simulink model "second_order_discrete"  (R2025b)
settings: Solver=VariableStepAuto  StartTime=0.0  StopTime=5  FixedStep=0.001  RelTol=1e-3
InitFcn:
  | % % Tunable knob
  | % T_set = 200;
  | % s_CL = -6/T_set;
  | % % Kp = s_CL^2;
  | % % Kd = -2*s_CL;
  | %
  | % % Kp = 0.001064;
  | % % Kd = 0.063514;
  | %
  | % % Kp = 0.000537;
  | % % Kd = 0.038196;
  | %
  | % % Kp = 0.00045;
  | % % Kd = 0.040196;
  | %
  | %             Kp = 0.0003;
  | %             Kd = 0.09;
  | %
  | % Kob = 10;
  | %
  | % %             K = 164.458741/50*1;
  | % % tau1 = 160.525043;
  | % % tau2 = 835.747525;
  | % %             L_comp = 13.297226;
  | % %             L_sys  = 13.297226;
  | % K = 1.467057642011806*2;
  | % K0 = 1.467057642011806*2;
  | % tau1 = 5.108331033027039e+02;
  | % tau2 = 35.728915073943433;
  | % L_comp = 15.024369999999999;
  | % L_sys = 15.024369999999999;
  | % % K = 1.455368;
  | % % K0 = 1.455368;
  | % % tau1 = 18.226428;
  | % % tau2 = 538.493088;
  | % % L_comp = 33.344271;
  | % % L_sys = 33.344271;
  | % t1 = tau1*tau2;
  | % b0 = K0/t1;
  | %
  | % % Derived quantities
  | % s_ESO = Kob*s_CL;
  | % l1 = -3*s_ESO;
  | % l2 = 3*s_ESO^2;
  | % l3 = -s_ESO^3;
  | %
  | % A = [-l1  1  0;
  | %      -l2  0  1
  | %      -l3  0  0];
  | %
  | % B = [0   l1
  | %      b0  l2;
  | %      0   l3];
  | %
  | % % discrete equivalent
  | % Ts = 0.005;
  | % Ad = [1  Ts  Ts^2/2
  | %       0   1      Ts
  | %       0   0       1];
  | % Bd = [b0*Ts^2/2; b0*Ts; 0];
  | % z_ESO = exp(s_ESO*Ts);
  | % dl1 = 1-z_ESO^3;
  | % dl2 = 3/(2*Ts) * (1-z_ESO)^2*(1+z_ESO);
  | % dl3 = 1/Ts^2 * (1-z_ESO)^3;
  | % Cd = [1 0 0]; Ld = [dl1;dl2;dl3];
  | % Aeso = Ad - Ld*Cd*Ad;
  | % Beso = Bd - Ld*Cd*Bd;
  | % delay_comp = round(L_comp*200);
  | % delay_sys  = round(L_sys*200);
  | % K1 = Kp; K2 = Kd;
  | 
  | 
  | 
  | % Tunable knob
  | T_set = 200;
  | s_CL = -6/T_set;
  | % Kp = s_CL^2;
  | % Kd = -2*s_CL;
  | Kp = 0.00055;
  | Kd = 0.06;
  | 
  | Kob = 2;
  | 
  | K = 1.6937;
  | K0 = 1.6937 ;
  | tau1 = 792.76;
  | tau2 = 56.103;
  | L_comp = 29.97;
  | L_sys = 29.97;
  | t1 = tau1*tau2;
  | b0 = K0/t1;
  | 
  | % Derived quantities
  | s_ESO = Kob*s_CL;
  | l1 = -3*s_ESO;
  | l2 = 3*s_ESO^2;
  | l3 = -s_ESO^3;
  | 
  | A = [-l1  1  0;
  |      -l2  0  1
  |      -l3  0  0];
  | 
  | B = [0   l1
  |      b0  l2;
  |      0   l3];
  | 
  | % discrete equivalent
  | Ts = 0.005;
  | Ad = [1  Ts  Ts^2/2
  |       0   1      Ts
  |       0   0       1];
  | Bd = [b0*Ts^2/2; b0*Ts; 0];
  | z_ESO = exp(s_ESO*Ts);
  | dl1 = 1-z_ESO^3;
  | dl2 = 3/(2*Ts) * (1-z_ESO)^2*(1+z_ESO);
  | dl3 = 1/Ts^2 * (1-z_ESO)^3;
  | Cd = [1 0 0]; Ld = [dl1;dl2;dl3];
  | Aeso = Ad - Ld*Cd*Ad;
  | Beso = Bd - Ld*Cd*Bd;
  | delay_comp = round(L_comp*200);
  | delay_sys  = round(L_sys*200);
  | K1 = Kp; K2 = Kd;
libraries: simulink_extras x1
settings Model: Creator=SARIR  LastModifiedBy=MG8102
settings RTWCC: GPUComputeCapability=3.5

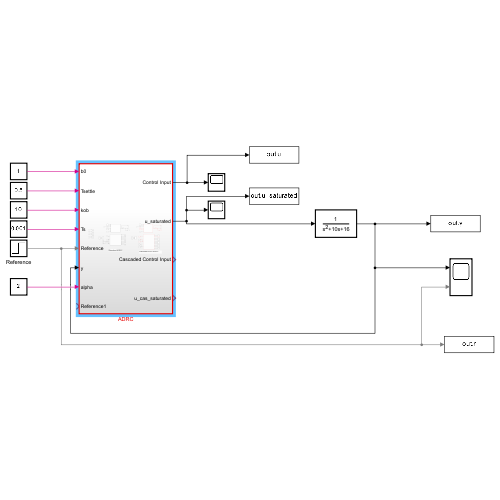
[thumbnail: Simulink's stored preview of the top-level diagram]
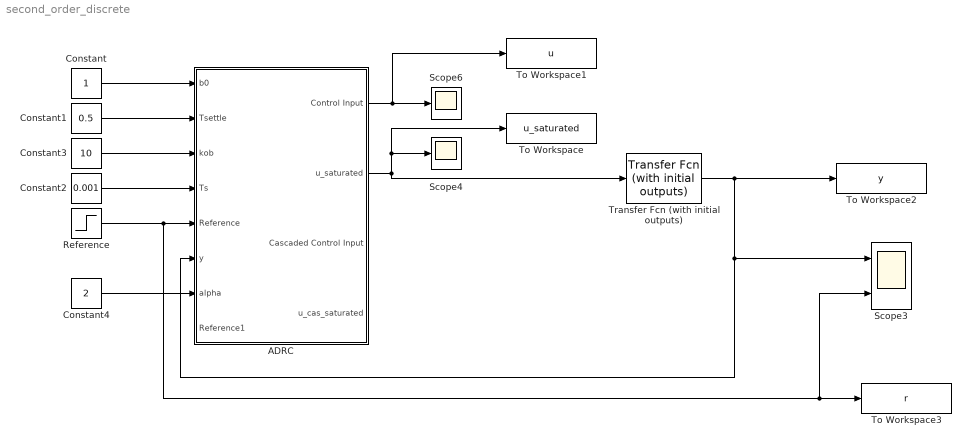
== system second_order_discrete ==
  ADRC : Subsystem
  Constant : Constant
  Constant1 : Constant  Value=0.5
  Constant2 : Constant  Value=0.001
  Constant3 : Constant  Value=10
  Constant4 : Constant  Value=2
  Reference : Step  Time=2  SampleTime=0
  Scope3 : Scope  NumInputPorts=2
      settings: ActiveDisplayYMinimum=-0.13260362865071351  ActiveDisplayYMaximum=1.1934326578564218
  Scope4 : Scope
      settings: ActiveDisplayYMinimum=-12.499999999999996  ActiveDisplayYMaximum=112.5  DataLoggingVariableName=ScopeData13
  Scope6 : Scope
      settings: ActiveDisplayYMinimum=-0.96663811924557952  ActiveDisplayYMaximum=8.8198546513386518  DataLoggingVariableName=ScopeData15
  To Workspace : ToWorkspace  VariableName=u_saturated  SaveFormat=Timeseries  SampleTime=-1
  To Workspace1 : ToWorkspace  VariableName=u  SaveFormat=Timeseries  SampleTime=-1
  To Workspace2 : ToWorkspace  VariableName=y  SaveFormat=Timeseries  SampleTime=-1
  To Workspace3 : ToWorkspace  VariableName=r  SaveFormat=Timeseries  SampleTime=-1
  Transfer Fcn (with initial outputs) : simulink_extras/Additional Linear/Transfer Fcn (with initial outputs)  N=[1]  D=[1 10 16]  Y0=0  U0=0
  wires:
  Reference/1 -> Scope3/2, To Workspace3/1, ADRC/5(Reference)
  Constant/1 -> ADRC/1(b0)
  Constant1/1 -> ADRC/2(Tsettle)
  Constant3/1 -> ADRC/3(kob)
  ADRC/1(Control Input) -> To Workspace1/1, Scope6/1
  ADRC/2(u_saturated) -> Scope4/1, To Workspace/1, Transfer Fcn (with initial outputs)/1
  Constant2/1 -> ADRC/4(Ts)
  Transfer Fcn (with initial outputs)/1 -> ADRC/6(y), Scope3/1, To Workspace2/1
  Constant4/1 -> ADRC/7(alpha)

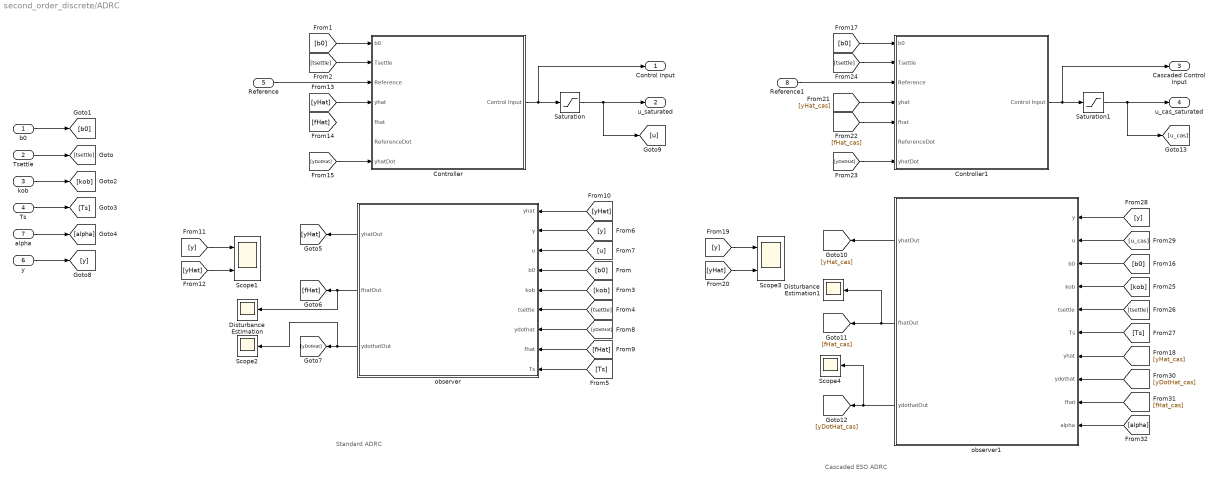
== system second_order_discrete/ADRC ==
  note: Standard ADRC
  note: Cascaded ESO ADRC
  b0 : Inport
  Tsettle : Inport  Port=2
  kob : Inport  Port=3
  Ts : Inport  Port=4
  Reference : Inport  Port=5
  y : Inport  Port=6
  alpha : Inport  Port=7
  Reference1 : Inport  Port=8
  Controller : Subsystem
  Controller1 : Subsystem
  Disturbance Estimation : Scope
      settings: ActiveDisplayYMinimum=-1  ActiveDisplayYMaximum=1  DataLoggingVariableName=ScopeData2
  Disturbance Estimation1 : Scope
      settings: ActiveDisplayYMinimum=-1  ActiveDisplayYMaximum=1  DataLoggingVariableName=ScopeData12
  Saturation : Saturate  UpperLimit=100  LowerLimit=0
  Saturation1 : Saturate  UpperLimit=100  LowerLimit=0
  Scope1 : Scope  NumInputPorts=2
      settings: ActiveDisplayYMinimum=-8.9116041220478586  ActiveDisplayYMaximum=80.204437098430745
  Scope2 : Scope
      settings: ActiveDisplayYMinimum=-1  ActiveDisplayYMaximum=1  DataLoggingVariableName=ScopeData2
  Scope3 : Scope  NumInputPorts=2
      settings: ActiveDisplayYMinimum=-8.9116041220478586  ActiveDisplayYMaximum=80.204437098430745  DataLoggingVariableName=ScopeData14
  Scope4 : Scope
      settings: ActiveDisplayYMinimum=-1  ActiveDisplayYMaximum=1  DataLoggingVariableName=ScopeData16
  observer : Subsystem
  observer1 : Subsystem
  Control Input : Outport
  u_saturated : Outport  Port=2
  Cascaded Control Input : Outport  Port=3
  u_cas_saturated : Outport  Port=4
  wires:
  Tsettle/1 -> [tsettle]
  [b0] -> Controller/1(b0)
  [tsettle] -> observer/6(tsettle)
  [kob] -> observer/5(kob)
  [b0] -> observer/4(b0)
  Controller/1(Control Input) -> Control Input/1, Saturation/1
  [tsettle] -> Controller/2(Tsettle)
  Saturation/1 -> [u], u_saturated/1
  Reference/1 -> Controller/3(Reference)
  kob/1 -> [kob]
  b0/1 -> [b0]
  [Ts] -> observer/9(Ts)
  Ts/1 -> [Ts]
  alpha/1 -> [alpha]
  observer/1(yhatOut) -> [yHat]
  observer/2(fhatOut) -> Disturbance Estimation/1, [fHat]
  observer/3(ydothatOut) -> Scope2/1, [yDotHat]
  y/1 -> [y]
  [y] -> observer/2(y)
  [yHat] -> observer/1(yhat)
  [yDotHat] -> observer/7(ydothat)
  [fHat] -> observer/8(fhat)
  [u] -> observer/3(u)
  [yHat] -> Scope1/2
  [y] -> Scope1/1
  [yHat] -> Controller/4(yhat)
  [yDotHat] -> Controller/7(yhatDot)
  [y] -> Scope3/1
  [yDotHat] -> Controller1/7(yhatDot)
  [yHat] -> Scope3/2
  [b0] -> Controller1/1(b0)
  Controller1/1(Control Input) -> Cascaded Control Input/1, Saturation1/1
  Reference1/1 -> Controller1/3(Reference)
  [yHat_cas] -> Controller1/4(yhat)
  Saturation1/1 -> [u_cas], u_cas_saturated/1
  [tsettle] -> Controller1/2(Tsettle)
  observer1/1(yhatOut) -> [yHat_cas]
  observer1/2(fhatOut) -> [fHat_cas], Disturbance Estimation1/1
  observer1/3(ydothatOut) -> Scope4/1, [yDotHat_cas]
  [fHat_cas] -> Controller1/5(fhat)
  [yHat_cas] -> observer1/7(yhat)
  [u_cas] -> observer1/2(u)
  [y] -> observer1/1(y)
  [b0] -> observer1/3(b0)
  [tsettle] -> observer1/5(tsettle)
  [kob] -> observer1/4(kob)
  [Ts] -> observer1/6(Ts)
  [yDotHat_cas] -> observer1/8(ydothat)
  [fHat_cas] -> observer1/9(fhat)
  [alpha] -> observer1/10(alpha)

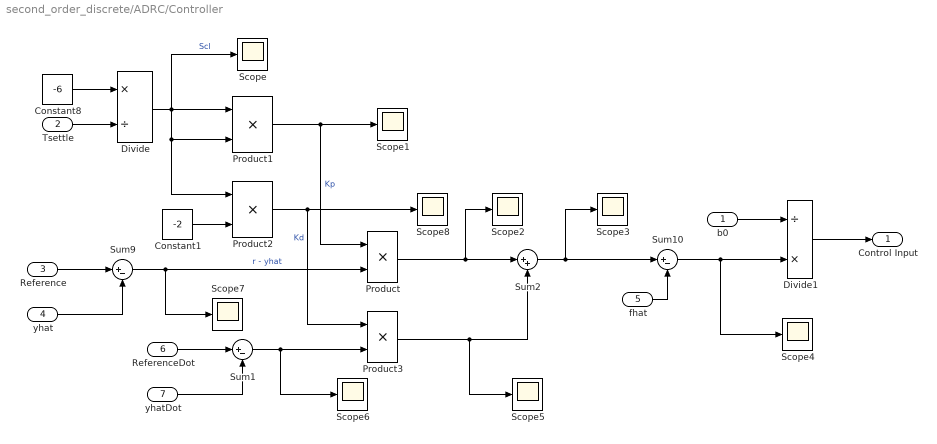
== system second_order_discrete/ADRC/Controller ==
  b0 : Inport
  Tsettle : Inport  Port=2
  Reference : Inport  Port=3
  yhat : Inport  Port=4
  fhat : Inport  Port=5
  ReferenceDot : Inport  Port=6
  yhatDot : Inport  Port=7
  Constant1 : Constant  Value=-2
  Constant8 : Constant  Value=-6
  Divide : Product  Inputs=*/
  Divide1 : Product  Inputs=/*
  Product{,1..3} (4 alike) : Product
  Scope{,1..8} (9 alike) : Scope
      Scope settings: ActiveDisplayYMinimum=-1  ActiveDisplayYMaximum=1  DataLoggingVariableName=ScopeData3
      Scope1 settings: ActiveDisplayYMinimum=-1  ActiveDisplayYMaximum=1  DataLoggingVariableName=ScopeData4
      Scope2 settings: ActiveDisplayYMinimum=-1  ActiveDisplayYMaximum=1  DataLoggingVariableName=ScopeData5
      Scope3 settings: ActiveDisplayYMinimum=-1  ActiveDisplayYMaximum=1  DataLoggingVariableName=ScopeData6
      Scope4 settings: ActiveDisplayYMinimum=-0.195  ActiveDisplayYMaximum=1.755  DataLoggingVariableName=ScopeData7
      Scope5 settings: ActiveDisplayYMinimum=-1  ActiveDisplayYMaximum=1  DataLoggingVariableName=ScopeData8
      Scope6 settings: ActiveDisplayYMinimum=-0.40718  ActiveDisplayYMaximum=1.15635  DataLoggingVariableName=ScopeData9
      Scope7 settings: ActiveDisplayYMinimum=-0.12554  ActiveDisplayYMaximum=1.12506  DataLoggingVariableName=ScopeData10
      Scope8 settings: ActiveDisplayYMinimum=0.2  ActiveDisplayYMaximum=2.2  DataLoggingVariableName=ScopeData11
  Sum1 : Sum  Inputs=|+-
  Sum10 : Sum  Inputs=|+-
  Sum2 : Sum  Inputs=|++
  Sum9 : Sum  Inputs=|+-
  Control Input : Outport
  wires:
  Divide1/1 -> Control Input/1
  Constant8/1 -> Divide/1
  Sum9/1 -> Scope7/1, Product/2  "r - yhat"
  yhat/1 -> Sum9/2
  Tsettle/1 -> Divide/2
  Sum10/1 -> Scope4/1, Divide1/2
  Reference/1 -> Sum9/1
  b0/1 -> Divide1/1
  fhat/1 -> Sum10/2
  Divide/1 -> Product2/1, Product1/2, Scope/1, Product1/1  "Scl"
  Product1/1 -> Scope1/1, Product/1  "Kp"
  ReferenceDot/1 -> Sum1/1
  yhatDot/1 -> Sum1/2
  Constant1/1 -> Product2/2
  Sum1/1 -> Scope6/1, Product3/2
  Product2/1 -> Scope8/1, Product3/1  "Kd"
  Sum2/1 -> Scope3/1, Sum10/1
  Product/1 -> Scope2/1, Sum2/1
  Product3/1 -> Scope5/1, Sum2/2

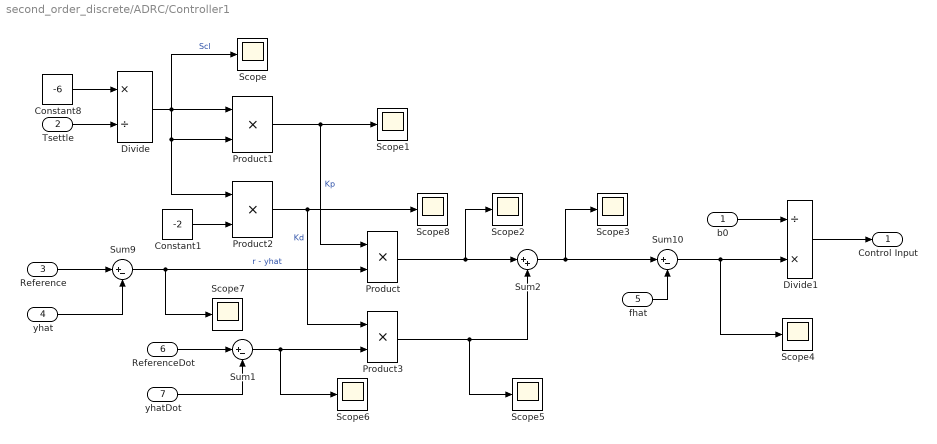
== system second_order_discrete/ADRC/Controller1 ==
  b0 : Inport
  Tsettle : Inport  Port=2
  Reference : Inport  Port=3
  yhat : Inport  Port=4
  fhat : Inport  Port=5
  ReferenceDot : Inport  Port=6
  yhatDot : Inport  Port=7
  Constant1 : Constant  Value=-2
  Constant8 : Constant  Value=-6
  Divide : Product  Inputs=*/
  Divide1 : Product  Inputs=/*
  Product{,1..3} (4 alike) : Product
  Scope{,1..8} (9 alike) : Scope
      Scope settings: ActiveDisplayYMinimum=-1  ActiveDisplayYMaximum=1  DataLoggingVariableName=ScopeData3
      Scope1 settings: ActiveDisplayYMinimum=-1  ActiveDisplayYMaximum=1  DataLoggingVariableName=ScopeData4
      Scope2 settings: ActiveDisplayYMinimum=-1  ActiveDisplayYMaximum=1  DataLoggingVariableName=ScopeData5
      Scope3 settings: ActiveDisplayYMinimum=-1  ActiveDisplayYMaximum=1  DataLoggingVariableName=ScopeData6
      Scope4 settings: ActiveDisplayYMinimum=-0.195  ActiveDisplayYMaximum=1.755  DataLoggingVariableName=ScopeData7
      Scope5 settings: ActiveDisplayYMinimum=-1  ActiveDisplayYMaximum=1  DataLoggingVariableName=ScopeData8
      Scope6 settings: ActiveDisplayYMinimum=-0.40718  ActiveDisplayYMaximum=1.15635  DataLoggingVariableName=ScopeData9
      Scope7 settings: ActiveDisplayYMinimum=-0.12554  ActiveDisplayYMaximum=1.12506  DataLoggingVariableName=ScopeData10
      Scope8 settings: ActiveDisplayYMinimum=0.2  ActiveDisplayYMaximum=2.2  DataLoggingVariableName=ScopeData11
  Sum1 : Sum  Inputs=|+-
  Sum10 : Sum  Inputs=|+-
  Sum2 : Sum  Inputs=|++
  Sum9 : Sum  Inputs=|+-
  Control Input : Outport
  wires:
  Divide1/1 -> Control Input/1
  Constant8/1 -> Divide/1
  Sum9/1 -> Scope7/1, Product/2  "r - yhat"
  yhat/1 -> Sum9/2
  Tsettle/1 -> Divide/2
  Sum10/1 -> Scope4/1, Divide1/2
  Reference/1 -> Sum9/1
  b0/1 -> Divide1/1
  fhat/1 -> Sum10/2
  Divide/1 -> Product2/1, Product1/2, Scope/1, Product1/1  "Scl"
  Product1/1 -> Scope1/1, Product/1  "Kp"
  ReferenceDot/1 -> Sum1/1
  yhatDot/1 -> Sum1/2
  Constant1/1 -> Product2/2
  Sum1/1 -> Scope6/1, Product3/2
  Product2/1 -> Scope8/1, Product3/1  "Kd"
  Sum2/1 -> Scope3/1, Sum10/1
  Product/1 -> Scope2/1, Sum2/1
  Product3/1 -> Scope5/1, Sum2/2

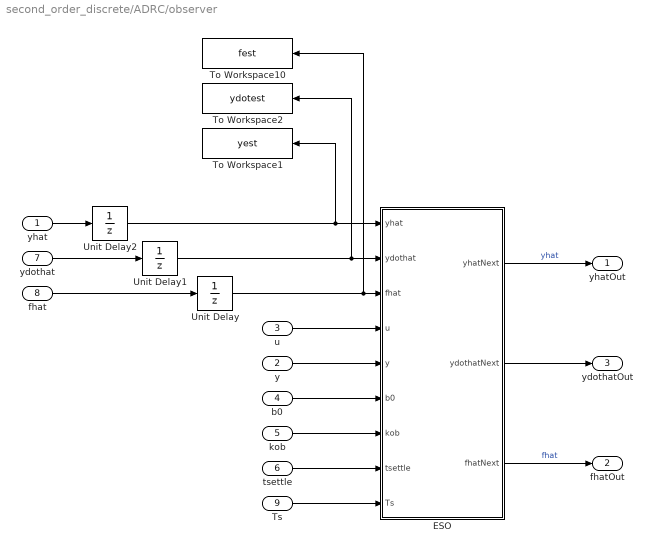
== system second_order_discrete/ADRC/observer ==
  yhat : Inport
  y : Inport  Port=2
  u : Inport  Port=3
  b0 : Inport  Port=4
  kob : Inport  Port=5
  tsettle : Inport  Port=6
  ydothat : Inport  Port=7
  fhat : Inport  Port=8
  Ts : Inport  Port=9
  ESO : MATLAB Function  TreatAsAtomicUnit=on
  To Workspace1 : ToWorkspace  VariableName=yest  SaveFormat=Timeseries  SampleTime=-1
  To Workspace10 : ToWorkspace  VariableName=fest  SaveFormat=Timeseries  SampleTime=-1
  To Workspace2 : ToWorkspace  VariableName=ydotest  SaveFormat=Timeseries  SampleTime=-1
  Unit Delay : UnitDelay  SampleTime=0.002  HasFrameUpgradeWarning=on
  Unit Delay1 : UnitDelay  SampleTime=0.002  HasFrameUpgradeWarning=on
  Unit Delay2 : UnitDelay  SampleTime=0.002  HasFrameUpgradeWarning=on
  yhatOut : Outport
  fhatOut : Outport  Port=2
  ydothatOut : Outport  Port=3
  wires:
  b0/1 -> ESO/6(b0)
  ESO/1(yhatNext) -> yhatOut/1  "yhat"
  kob/1 -> ESO/7(kob)
  yhat/1 -> Unit Delay2/1
  tsettle/1 -> ESO/8(tsettle)
  u/1 -> ESO/4(u)
  y/1 -> ESO/5(y)
  ESO/3(fhatNext) -> fhatOut/1  "fhat"
  ydothat/1 -> Unit Delay1/1
  fhat/1 -> Unit Delay/1
  ESO/2(ydothatNext) -> ydothatOut/1
  Ts/1 -> ESO/9(Ts)
  Unit Delay2/1 -> To Workspace1/1, ESO/1(yhat)
  Unit Delay1/1 -> To Workspace2/1, ESO/2(ydothat)
  Unit Delay/1 -> To Workspace10/1, ESO/3(fhat)

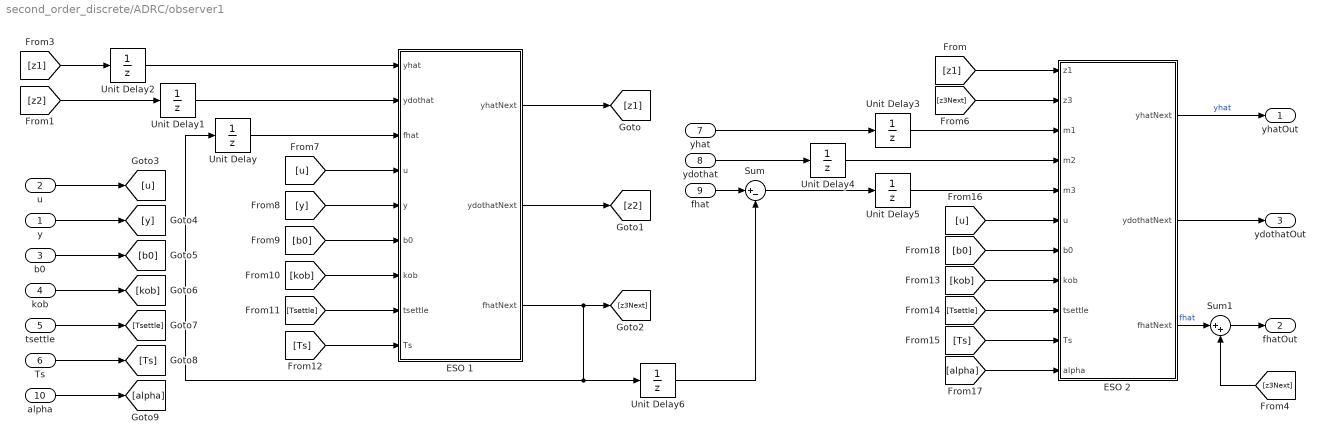
== system second_order_discrete/ADRC/observer1 ==
  y : Inport
  u : Inport  Port=2
  b0 : Inport  Port=3
  kob : Inport  Port=4
  tsettle : Inport  Port=5
  Ts : Inport  Port=6
  yhat : Inport  Port=7
  ydothat : Inport  Port=8
  fhat : Inport  Port=9
  alpha : Inport  Port=10
  ESO 1 : MATLAB Function  TreatAsAtomicUnit=on
  ESO 2 : MATLAB Function  TreatAsAtomicUnit=on
  Sum : Sum  Inputs=|+-
  Sum1 : Sum  Inputs=|++
  Unit Delay{,1..6} (7 alike) : UnitDelay  SampleTime=0.002  HasFrameUpgradeWarning=on
  yhatOut : Outport
  fhatOut : Outport  Port=2
  ydothatOut : Outport  Port=3
  wires:
  ESO 1/1(yhatNext) -> [z1]
  ESO 1/2(ydothatNext) -> [z2]
  Unit Delay2/1 -> ESO 1/1(yhat)
  Unit Delay1/1 -> ESO 1/2(ydothat)
  Unit Delay/1 -> ESO 1/3(fhat)
  ESO 2/2(ydothatNext) -> ydothatOut/1
  ESO 2/1(yhatNext) -> yhatOut/1  "yhat"
  Unit Delay3/1 -> ESO 2/3(m1)
  [z1] -> Unit Delay2/1
  ESO 1/3(fhatNext) -> Unit Delay6/1, Unit Delay/1, [z3Next]
  [z2] -> Unit Delay1/1
  [z1] -> ESO 2/1(z1)
  Sum/1 -> Unit Delay5/1
  fhat/1 -> Sum/1
  Unit Delay4/1 -> ESO 2/4(m2)
  Unit Delay5/1 -> ESO 2/5(m3)
  ESO 2/3(fhatNext) -> Sum1/1  "fhat"
  Sum1/1 -> fhatOut/1
  [z3Next] -> Sum1/2
  ydothat/1 -> Unit Delay4/1
  yhat/1 -> Unit Delay3/1
  [z3Next] -> ESO 2/2(z3)
  u/1 -> [u]
  y/1 -> [y]
  b0/1 -> [b0]
  kob/1 -> [kob]
  tsettle/1 -> [Tsettle]
  Ts/1 -> [Ts]
  [Ts] -> ESO 1/9(Ts)
  [Tsettle] -> ESO 1/8(tsettle)
  [kob] -> ESO 1/7(kob)
  [b0] -> ESO 1/6(b0)
  [y] -> ESO 1/5(y)
  [u] -> ESO 1/4(u)
  [u] -> ESO 2/6(u)
  [b0] -> ESO 2/7(b0)
  [Tsettle] -> ESO 2/9(tsettle)
  [kob] -> ESO 2/8(kob)
  [Ts] -> ESO 2/10(Ts)
  [alpha] -> ESO 2/11(alpha)
  alpha/1 -> [alpha]
  Unit Delay6/1 -> Sum/2

== matlab function second_order_discrete/ADRC/observer1/ESO 1 ==
  data: yhat input; ydothat input; fhat input; u input; yhatNext output; ydothatNext output; y input; b0 input; kob input; tsettle input; fhatNext output; Ts input
function [yhatNext, ydothatNext, fhatNext] = fcn(yhat, ydothat, fhat, u, y, b0, kob, tsettle, Ts)
    Kp = 6/tsettle;
    Scl = -Kp;
    Seso = kob * Scl;
    Zeso = exp(Seso * Ts);

    l1 = 1 - (Zeso)^3;
    l2 = (3 / (2 * Ts)) * ((1 - Zeso)^2) * (1 + Zeso);
    l3 = (1 / (Ts^2)) * ((1 - Zeso)^3);
    
    Ad = [1, Ts, (Ts^2)/2; 0, 1, Ts; 0, 0, 1]; 
    Bd = [b0*(Ts^2)/2; b0*Ts; 0];
    Cd = [1, 0, 0];
    Dd = 0;
    Ld = [l1; l2; l3];

    xPrev = [yhat; ydothat; fhat]; 
    xNext = (Ad - Ld*Cd*Ad) * xPrev + (Bd - Ld*Cd*Bd) * u + Ld * y;
     
    yhatNext = xNext(1);
    ydothatNext = xNext(2);
    fhatNext = xNext(3);

== matlab function second_order_discrete/ADRC/observer/ESO ==
  data: yhat input; ydothat input; fhat input; u input; yhatNext output; ydothatNext output; y input; b0 input; kob input; tsettle input; fhatNext output; Ts input
function [yhatNext, ydothatNext, fhatNext] = fcn(yhat, ydothat, fhat, u, y, b0, kob, tsettle, Ts)
    Kp = 6/tsettle;
    Scl = -Kp;
    Seso = kob * Scl;
    Zeso = exp(Seso * Ts);

    l1 = 1 - (Zeso)^3;
    l2 = (3 / (2 * Ts)) * ((1 - Zeso)^2) * (1 + Zeso);
    l3 = (1 / (Ts^2)) * ((1 - Zeso)^3);
    
    Ad = [1, Ts, (Ts^2)/2; 0, 1, Ts; 0, 0, 1]; 
    Bd = [b0*(Ts^2)/2; b0*Ts; 0];
    Cd = [1, 0, 0];
    Dd = 0;
    Ld = [l1; l2; l3];

    xPrev = [yhat; ydothat; fhat]; 
    xNext = (Ad - Ld*Cd*Ad) * xPrev + (Bd - Ld*Cd*Bd) * u + Ld * y;
     
    yhatNext = xNext(1);
    ydothatNext = xNext(2);
    fhatNext = xNext(3);

== matlab function second_order_discrete/ADRC/observer1/ESO 2 ==
  data: z1 input; z3 input; m1 input; m2 input; m3 input; u input; yhatNext output; ydothatNext output; b0 input; kob input; tsettle input; fhatNext output; Ts input; alpha input
function [yhatNext, ydothatNext, fhatNext] = fcn(z1, z3, m1, m2, m3, u, b0, kob, tsettle, Ts, alpha)
    Kp = 6/tsettle;
    Scl = -Kp;
    Seso = kob * Scl * alpha;
    Zeso = exp(Seso * Ts);

    l1 = 1 - (Zeso)^3;
    l2 = (3 / (2 * Ts)) * ((1 - Zeso)^2) * (1 + Zeso);
    l3 = (1 / (Ts^2)) * ((1 - Zeso)^3);
    
    Ad = [1, Ts, (Ts^2)/2; 0, 1, Ts; 0, 0, 1]; 
    Bd = [b0*(Ts^2)/2; b0*Ts; 0];
    Cd = [1, 0, 0];
    Dd = 0;
    Ld = [l1; l2; l3];

    xPrev = [m1; m2; m3]; 
    xNext = (Ad - Ld*Cd*Ad) * xPrev + (Bd - Ld*Cd*Bd) * u + Ld * z1 + z3;
     
    yhatNext = xNext(1);
    ydothatNext = xNext(2);
    fhatNext = xNext(3);
